simulink model "Model_verification_external"  (R2013b)
settings: Solver=FixedStepDiscrete  SolverMode=SingleTasking  StartTime=0.0  StopTime=4  FixedStep=sim_step_size  RelTol=1e-3
PreLoadFcn:
  | motor_parameters;
InitFcn:
  | Vref = 4.5; % Run in external mode
  | LoopGain = 0.12;
  | 
  | % Controller parameters
  | Kp = 0.9;
  | Ki = 38;
  | Kd = 0;
  | 
  | % Simulation parameters
  | % sim_stop_time = 4; % period of pulse is 4 seconds
  | sim_step_size = 0.01; % 0.001;
  | ctl_step_size = 0.03;
values from neighbouring files (symbols this model uses):
  Counts2RAD = 0.00872664625997    [Ideal_2ndOrder_PI_Prop_only.mat]    (also in Ideal_2ndOrder_PI_Sat.mat; Ideal_2ndOrder_PI_Sat_CtlStep.mat; Ideal_2ndOrder_PI_Sat_CtlStep_Q.mat; Ideal_2ndOrder_PI_Sat_CtlStep_Q_verification.mat)
libraries: simulink x2
settings Model: SimulationMode=external  ExtModeTrigDuration=2  Creator=nding  LastModifiedBy=nding
settings OptimizationCC: OptimizeModelRefInitCode=on  LifeSpan=1
settings DebuggingCC: SolverPrmCheckMsg=none
settings HardwareCC: ProdBitPerInt=16  ProdBitPerPointer=8  ProdIntDivRoundTo=Zero  ProdEndianess=LittleEndian  ProdWordSize=8  ProdHWDeviceType=Atmel->AVR
settings RTWCC: SystemTargetFile=realtime.tlc  GenerateMakefile=off  TemplateMakefile=realtime.tmf  Description=Run on Target Hardware  RTWVerbose=off  ProcessScript=realtime_make_rtw_hook
settings STFCustomTargetCC: TargetLibSuffix=.a  GenerateSampleERTMain=on  ERTCustomFileBanners=on  SupportNonInlinedSFcns=off  SupportVariableSizeSignals=on  MATLABClassNameForMDSCustomization=Simulink.SoftwareTarget.ERTCustomization  GRTInterface=off  SystemTargetFile=realtime.tlc
settings ERTTargetCC: CodeReplacementLibrary=ANSI_C  GenerateSampleERTMain=on  ParMdlRefBuildCompliant=off  CompOptLevelCompliant=off  ConcurrentExecutionCompliant=off  CombineOutputUpdateFcns=off  ERTFirstTimeCompliant=off  SupportContinuousTime=on  SupportVariableSizeSignals=on  ModelStepFunctionPrototypeControlCompliant=off  CPPClassGenCompliant=off  ExtModeTransport=3  ExtModeMexFile=ext_serial_win32_comm  ExtModeMexArgs=0 1 9600  InlinedParameterPlacement=NonHierarchical  ERTSrcFileBannerTemplate=realtime_code_template.cgt  ERTHdrFileBannerTemplate=realtime_code_template.cgt  ERTDataSrcFileTemplate=realtime_code_template.cgt  ERTDataHdrFileTemplate=realtime_code_template.cgt  ERTCustomFileTemplate=realtime_file_process.tlc

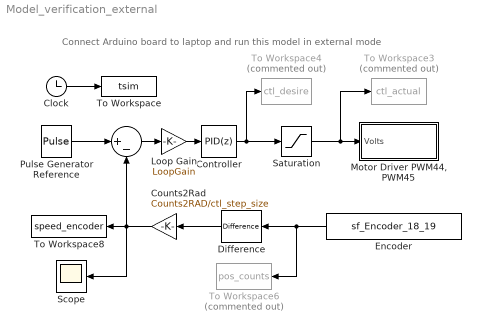
== system Model_verification_external ==
  note: Connect Arduino board to laptop and run this model in external mode
  " " : Sum  Inputs=|+-
  Clock : Clock
  Controller : simulink/Continuous/PID Controller  Controller=PID  TimeDomain=Discrete-time  SampleTime=ctl_step_size  IntegratorMethod=Forward Euler  FilterMethod=Forward Euler  Form=Parallel  P=Kp  I=Ki  D=0  N=100  InitialConditionSource=internal  InitialConditionForIntegrator=0  InitialConditionForFilter=0  ExternalReset=none  LimitOutput=off  UpperSaturationLimit=inf  LowerSaturationLimit=-inf  LinearizeAsGain=off  AntiWindupMode=none  Kb=1  TrackingMode=off  Kt=1  PParamMin=[]  PParamMax=[]  IParamMin=[]  IParamMax=[]  DParamMin=[]  DParamMax=[]  NParamMin=[]  NParamMax=[]  KbParamMin=[]  KbParamMax=[]  KtParamMin=[]  KtParamMax=[]  POutMin=[]  POutMax=[]  IOutMin=[]  IOutMax=[]  DOutMin=[]  DOutMax=[]  NOutMin=[]  NOutMax=[]  KbOutMin=[]  KbOutMax=[]  KtOutMin=[]  KtOutMax=[]  IntegratorOutMin=[]  IntegratorOutMax=[]  FilterOutMin=[]  FilterOutMax=[]  SumOutMin=[]  SumOutMax=[]  SumI1OutMin=[]  SumI1OutMax=[]  SumI2OutMin=[]  SumI2OutMax=[]  SumI3OutMin=[]  SumI3OutMax=[]  SumDOutMin=[]  SumDOutMax=[]  SaturationOutMin=[]  SaturationOutMax=[]  IntegratorContinuousStateAttributes=''  IntegratorStateMustResolveToSignalObject=off  IntegratorRTWStateStorageClass=Auto  FilterContinuousStateAttributes=''  FilterStateMustResolveToSignalObject=off  FilterRTWStateStorageClass=Auto
  Counts2Rad : Gain  Gain=Counts2RAD/ctl_step_size  OutDataTypeStr=double
  Difference : simulink/Discrete/Difference  ICPrevInput=0.0  InputProcessing=Inherited  OutMin=[]  OutMax=[]  OutDataType=fixdt(1, 16)  OutScaling=2^-10  DoSatur=off
  Encoder : S-Function  InitFcn=try, set_param(gcb,'FunctionName','sf_Encoder_18_19'), end  FunctionName=sf_Encoder_18_19  Parameters=uint8(0),uint8(18),uint8(19)  SFunctionModules=sf_Encoder_18_19_wrapper  EnableBusSupport=off  mask(S-Function Builder){}
      mask init:
      | val = [[.9  0.75 0.75 1 1 .9 .9 1]',[1 1 0.75 0.75 .9 .9 1 .9]'];try , sys = get_param(gcb,'SfunBuilderFcnName');if isempty(sys), sys = get_param(gcb,'FunctionName'); end,catch, sys = get_param(gcb,'FunctionName'); end
      settings: CopyFcn=set_param(gcbh,'LinkStatus','none')  PreSaveFcn=try, set_param(gcb,'FunctionName','sf_Encoder_18_19'), end  OpenFcn=sfunctionwizard(gcbh)
      mask Display: plot(val(:,1),val(:,2)),disp(sys), port_label('output',1,'pos')
  Loop Gain : Gain  Gain=LoopGain
  "Motor Driver PWM44, PWM45" : Subsystem  mask{Vs=Vref, Delta=0}
      mask prompts: Vs "Supply Voltage Vs: USB 4.5v; Battery 9v"; Delta "PWM Offset Delta: 0-255"
      mask init:
      | Vusb=4.5;
      | Vbat=9.0;
      mask DialogControl T Prompt: Specify Motor Supply Voltage and PWM Offset
  Pulse Generator Reference : DiscretePulseGenerator  PulseType=Time based  Amplitude=3.14  PulseWidth=50  SampleTime=sim_step_size
  Saturation : Saturate  UpperLimit=Vref  LowerLimit=-Vref
  Scope : Scope
      settings: YMin=0  YMax=6.5
  To Workspace : ToWorkspace  VariableName=tsim  SampleTime=sim_step_size
  To Workspace3 : ToWorkspace  Commented=on  VariableName=ctl_actual  SampleTime=sim_step_size
  To Workspace4 : ToWorkspace  Commented=on  VariableName=ctl_desire  SampleTime=sim_step_size
  To Workspace6 : ToWorkspace  Commented=on  VariableName=pos_counts  SampleTime=sim_step_size
  To Workspace8 : ToWorkspace  VariableName=speed_encoder  SampleTime=sim_step_size
  wires:
  Clock/1 -> To Workspace/1
  Pulse Generator Reference/1 -> " "/1
  Controller/1 -> Saturation/1, To Workspace4/1
  Loop Gain/1 -> Controller/1
  " "/1 -> Loop Gain/1
  Saturation/1 -> "Motor Driver PWM44, PWM45"/1(Volts), To Workspace3/1
  Encoder/1 -> To Workspace6/1, Difference/1
  Difference/1 -> Counts2Rad/1
  Counts2Rad/1 -> Scope/1, To Workspace8/1, " "/2

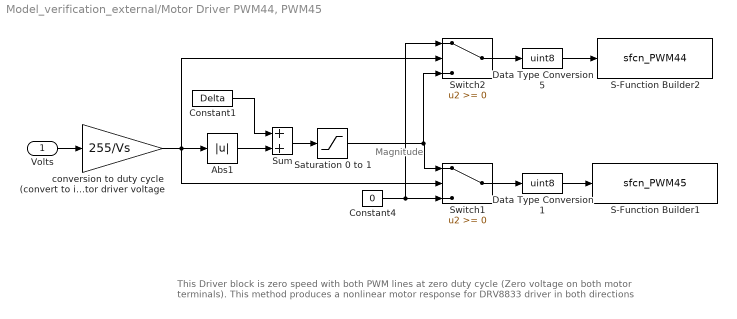
== system Model_verification_external/Motor Driver PWM44, PWM45 ==
  note: Magnitude
  note: This Driver block is zero speed with both PWM lines at zero duty cycle  (Zero voltage on both motor terminals).
      | This method produces a nonlinear motor response for DRV8833 driver in both directions
  Volts : Inport
  Abs1 : Abs
  Constant1 : Constant  Value=Delta
  Constant4 : Constant  Value=0
  Data Type Conversion1 : DataTypeConversion  OutDataTypeStr=uint8
  Data Type Conversion5 : DataTypeConversion  OutDataTypeStr=uint8
  S-Function Builder1 : S-Function  InitFcn=try, set_param(gcb,'FunctionName','sfcn_PWM45'), end  FunctionName=sfcn_PWM45  Parameters=uint8(45)  SFunctionModules=sfcn_PWM45_wrapper  EnableBusSupport=off  mask(S-Function Builder){}
      mask init: same as Model_verification_external/Encoder
      settings: CopyFcn=set_param(gcbh,'LinkStatus','none')  PreSaveFcn=try, set_param(gcb,'FunctionName','sfcn_PWM45'), end  OpenFcn=sfunctionwizard(gcbh)
      mask Display: plot(val(:,1),val(:,2)),disp(sys), port_label('input',1,'in')
  S-Function Builder2 : S-Function  InitFcn=try, set_param(gcb,'FunctionName','sfcn_PWM44'), end  FunctionName=sfcn_PWM44  Parameters=uint8(44)  SFunctionModules=sfcn_PWM44_wrapper  EnableBusSupport=off  mask(S-Function Builder){}
      mask init: same as Model_verification_external/Encoder
      settings: CopyFcn=set_param(gcbh,'LinkStatus','none')  PreSaveFcn=try, set_param(gcb,'FunctionName','sfcn_PWM44'), end  OpenFcn=sfunctionwizard(gcbh)
      mask Display: plot(val(:,1),val(:,2)),disp(sys), port_label('input',1,'in')
  Saturation 0 to 1 : Saturate  UpperLimit=255  LowerLimit=0
  Sum : Sum
  Switch1 : Switch
  Switch2 : Switch
  conversion to duty cycle (convert to int) denominator is motor driver voltage : Gain  Gain=255/Vs  OutDataTypeStr=int16
  wires:
  Constant1/1 -> Sum/1
  Sum/1 -> Saturation 0 to 1/1
  Abs1/1 -> Sum/2
  Data Type Conversion1/1 -> S-Function Builder1/1
  Data Type Conversion5/1 -> S-Function Builder2/1
  Switch1/1 -> Data Type Conversion1/1
  Switch2/1 -> Data Type Conversion5/1
  Saturation 0 to 1/1 -> Switch1/1, Switch2/3
  Constant4/1 -> Switch1/3, Switch2/1
  conversion to duty cycle (convert to int) denominator is motor driver voltage/1 -> Switch2/2, Abs1/1, Switch1/2
  Volts/1 -> conversion to duty cycle (convert to int) denominator is motor driver voltage/1
